simulink model "ADCSSimulator"  (R2024a)
settings: Solver=ode4  StartTime=0.0  StopTime=600  FixedStep=0.01  MaxStep=0.1  RelTol=1e-3  AbsTol=1e-3
values from neighbouring files (symbols this model uses):
  ActuatorAllocationMatrix = ActuatorPhysicalMatrix' * inv(ActuatorPhysicalMatrix * ActuatorPhysicalMatrix')    [set_Init.m]
  ActuatorPhysicalMatrix = [1, 0, 0, 0 ... (first row only)    [set_Init.m]
  albedo_irradiance = 300    [set_Init.m]
  b = 0    [set_Init.m]
  Cd = 2.2    [set_Init.m]
  h_bias = [0; 0; 0]    [set_Init.m]
  J = 4.0e-3 / 628    (= 6.36942675159e-06)    [set_Init.m]
  k_Bdot = ((4 * pi * 0.5236 * 0.0055) / (5677.2 * (4.5e-5)^2))    (= 3147.8423197)    [set_Init.m]
  K_E = K_T    (= 0.0022)    [set_Init.m]
  K_T = 0.0022    [set_Init.m]
  P0 = blkdiag(P0_att, P0_bias)    [set_Init.m]
  P0_att = eye(3) * initial_variance_rad2    [set_Init.m]
  PowerVoltageBus_01 = 3.3    [set_Init.m]
  PowerVoltageBus_02 = 3.3    [set_Init.m]
  PowerVoltageBus_03 = 3.3    [set_Init.m]
  PowerVoltageBus_04 = 3.3    [set_Init.m]
  PowerVoltageBus_05 = 3.3    [set_Init.m]
  PowerVoltageBus_06 = 3.3    [set_Init.m]
  PowerVoltageBus_07 = 3.3    [set_Init.m]
  PowerVoltageBus_08 = 3.3    [set_Init.m]
  PowerVoltageBus_09 = 3.3    [set_Init.m]
  PowerVoltageBus_10 = 3.3    [set_Init.m]
  PowerVoltageBus_11 = 3.3    [set_Init.m]
  PowerVoltageBus_12 = 0.0    (= 0)    [set_Init.m]
  PowerVoltageBus_13 = 0.0    (= 0)    [set_Init.m]
  PowerVoltageBus_14 = 0.0    (= 0)    [set_Init.m]
  PowerVoltageBus_15 = 0.0    (= 0)    [set_Init.m]
  R = 2.0    (= 2)    [set_Init.m]
  ressidual_m = [3e-4; -2e-4; 1e-4]    [set_Init.m]
  solar_irradiance = 1361    [set_Init.m]
  surface_areas = [A_xy, A_yz, A_xz, A_xy, A_yz, A_xz]    [set_Init.m]
  surface_normals_body = [eye(3) -eye(3)]    [set_Init.m]
  surface_positions_body = [       hx,   0,   0 ... (first row only)    [set_Init.m]
  surface_reflectivities = [0.9 0.8 0.9 0.9 0.9 0.9]    [set_Init.m]
  Switch_01 = 1    [set_Init.m]
  Switch_02 = 1    [set_Init.m]
  Switch_03 = 1    [set_Init.m]
  Switch_04 = 1    [set_Init.m]
  Switch_05 = 1    [set_Init.m]
  Switch_06 = 1    [set_Init.m]
  Switch_07 = 1    [set_Init.m]
  Switch_08 = 1    [set_Init.m]
  Switch_09 = 1    [set_Init.m]
  Switch_10 = 1    [set_Init.m]
  Switch_11 = 1    [set_Init.m]
  Switch_12 = 0    [set_Init.m]
  Switch_13 = 0    [set_Init.m]
  Switch_14 = 0    [set_Init.m]
  Switch_15 = 0    [set_Init.m]
  visSampleTime = 0.1    [set_Init.m]
undefined symbols (not defined in the file or in its folder): attitude, Controller, epoch, IAU, juliandate, Kd, km, Kp, m, rad, s, satellite, SGP4_parameters, simulator, UKF_parameters, WMM2020
libraries: sharedtransform x27, aerolibutil x22, aerolibconvert2 x18, simulink_extras x16, matrix_library x6, aerolibtransform2 x4, vrlib x2, aerolibgravity2 x2, aerolibobsolete x1, aerolibattitudesys x1, simulink x1
(part 3 of 8)

== system ADCSSimulator/ADCS/ADCS Hardware/Actuators/Tri-axial Magnetorquer Model (MTQs) ==
  Magnetic Field [Body] (T) : Inport
  MTQ CMD (A.m^2) : Inport  Port=2  PortDimensions=[3,1]
  Bus Voltage : Inport  Port=3
  Abs : Abs  SaturateOnIntegerOverflow=off
  Abs1 : Abs  SaturateOnIntegerOverflow=off
  Bus Creator : BusCreator  Inputs=3
  Bus Selector : BusSelector  OutputSignals=Power Bus: MTQ_X (signal 9),Power Bus: MTQ_Y (signal 10),Power Bus: MTQ_Z (signal 11)
  Constant : Constant  Value=[1;1;1]
  Constant1 : Constant  Value=[1;1;1]
  Cross Product : vrlib/Utilities/Cross Product
  Demux : Demux  Outputs=3
  Gain : Gain  Gain=0.5
  Gain1 : Gain  Gain=-1
  Gain2 : Gain  Gain=0.5
  Magnetorquers Bus Creator : BusCreator  Inputs=3
  Mux : Mux  Inputs=3
  Nominal Dipole : Constant  Value=satellite.MTQ.DPMoment
  Power Consumption Calculator : Subsystem
  Power Consumption Calculator1 : Subsystem
  Power Consumption Calculator2 : Subsystem
  Product : Product  Inputs=3
  Product1 : Product  Inputs=*/
  Product2 : Product
  Product3 : Product
  Sign{,1..3} (4 alike) : Signum
  Sum : Sum  Inputs=|+-
  Sum1 : Sum  Inputs=|++
  Sum2 : Sum  Inputs=|++
  Sum3 : Sum  Inputs=|++
  maximum allowable magnetic dipole moment : Constant  Value=satellite.MTQ.DPMoment
  Acutators: MTQs : Outport
  wires:
  Product3/1 -> Abs/1, Product2/1, Sign1/1, Product1/1  "m_mod"
  Product2/1 -> Sum3/1
  Product1/1 -> Abs1/1
  Gain/1 -> Product/2  "1: |m_mod| > m_max"
  Abs1/1 -> Demux/1
  Product/1 -> Sum3/2
  Sum1/1 -> Gain/1  "2: |m_mod| > m_max"
  Nominal Dipole/1 -> Sum/2, Product/3  "m_max"
  Sign/1 -> Sum1/1  "1: |m_mod| > m_max"
  Bus Creator/1 -> Magnetorquers Bus Creator/3  "MTQs Power Status"
  Magnetic Field [Body] (T)/1 -> Cross Product/2
  Gain2/1 -> Product2/2  "1: m_max > |m_mod|"
  Sum3/1 -> Magnetorquers Bus Creator/1, Cross Product/1  "Dipoles (Am^2)"
  maximum allowable magnetic dipole moment/1 -> Product1/2
  Sum2/1 -> Gain2/1  "2: m_max > |m_mod|"
  Sign2/1 -> Sum2/1  "1: m_max > |m_mod|"
  Constant1/1 -> Sum2/2
  Sum/1 -> Gain1/1, Sign/1
  MTQ CMD (A.m^2)/1 -> Product3/1
  Magnetorquers Bus Creator/1 -> Acutators: MTQs/1  "Actuators"
  Constant/1 -> Sum1/2
  Cross Product/1 -> Magnetorquers Bus Creator/2  "MTQs Torque [Body] (Nm)"
  Sign1/1 -> Product/1
  Gain1/1 -> Sign2/1  "m_max - |m_mod|"
  Abs/1 -> Sum/1  "|m_mod|"
  Power Consumption Calculator2/1(Power Consumption) -> Bus Creator/1  "Power Consumption [Magnetorquer X]"
  Power Consumption Calculator/1(Power Consumption) -> Bus Creator/3  "Power Consumption [Magnetorquer Z]"
  Power Consumption Calculator1/1(Power Consumption) -> Bus Creator/2  "Power Consumption [Magnetorquer Y]"
  Sign3/1 -> Product3/2  "MTQ Switches"
  [InputVoltage] -> Sign3/1
  Demux/1 -> [DipoleRatioX]  "|m/m_max| (X)"
  Demux/2 -> [DipoleRatioY]  "|m/m_max| (Y)"
  Demux/3 -> [DipoleRatioZ]  "|m/m_max| (Z)"
  [DipoleRatioX] -> Power Consumption Calculator2/2(|m/m_max|)
  [DipoleRatioY] -> Power Consumption Calculator1/2(|m/m_max|)
  [DipoleRatioZ] -> Power Consumption Calculator/2(|m/m_max|)
  Bus Voltage/1 -> Bus Selector/1
  Mux/1 -> [InputVoltage]
  Bus Selector/1 -> Mux/1, Power Consumption Calculator2/1(Bus Voltage (V))  "<Power Bus: MTQ_X (signal 9)>"
  Bus Selector/2 -> Mux/2, Power Consumption Calculator1/1(Bus Voltage (V))  "<Power Bus: MTQ_Y (signal 10)>"
  Bus Selector/3 -> Mux/3, Power Consumption Calculator/1(Bus Voltage (V))  "<Power Bus: MTQ_Z (signal 11)>"

== system ADCSSimulator/ADCS/ADCS Hardware/Sensors/Analog Magnetometer Model ==
  note: sensivity is used for analog magnetometer
  Magnetic Field [Body] (T) : Inport
  Temperature (˚C) : Inport  Port=2
  Input Voltage (V) : Inport  Port=3
  Measurement Model DCM : Inport  Port=4
  Constant1 : Constant  Value=[1e-4, 1e-4,1e-4]
  Gain3 : Gain  Gain=10^-9
  Init Data Wrapper : Subsystem
  MATLAB Function : MATLAB Function  Commented=on  TreatAsAtomicUnit=on
  Matrix Multiply : Product  Multiplication=Matrix(*)
  Noise : RandomNumber  Variance=satellite.MM.NoiseVariance  SampleTime=1/satellite.MM.Frequency
  Nominal Temperature (˚C) : Constant  Value=20
  Offset (nT) : Constant  Value=satellite.MM.ZeroFieldBias*satellite.MM.Sensitivity
  Power Consumption Calculator : Subsystem
  Product : Product  Inputs=3
  Product1 : Product
  Product2 : Product
  Product4 : Product
  Quantization : Quantizer  QuantizationInterval=satellite.MM.QuantizationInterval
  Saturation : Saturate  UpperLimit=satellite.MM.Range(2)  LowerLimit=satellite.MM.Range(1)
  Scale Factor Drift : Constant  Value=satellite.MM.ScaleFactorDrift*1e-6
  Scale error : Constant  Value=satellite.MM.Accuracy*1e-2
  Sensivity : Gain  Gain=satellite.MM.Sensitivity
  Sign : Signum
  Sum : Sum  Inputs=+++++
  Sum1 : Sum  Inputs=++|
  Sum2 : Sum  Inputs=|+-
  Sum3 : Sum  Inputs=++|
  T to nT : Gain  Gain=10^9
  Unit Delay4 : UnitDelay  SampleTime=-1  HasFrameUpgradeWarning=on
  Zero Field Bias (nT) : Constant  Value=satellite.MM.ZeroFieldBias
  Zero Field Drift : Constant  Value=satellite.MM.ZeroFieldDrift
  Zero-Order Hold : ZeroOrderHold  SampleTime=1/satellite.MM.Frequency
  Measured Magnetic Field [Body] (T) : Outport  PortDimensions=[3,1]
  Power Consumption : Outport  Port=2
  wires:
  Zero Field Bias (nT)/1 -> Sum3/1
  T to nT/1 -> Sum3/2
  Quantization/1 -> Init Data Wrapper/1(Real Data)
  Init Data Wrapper/1(Wrapped Data) -> Measured Magnetic Field [Body] (T)/1
  Constant1/1 -> Init Data Wrapper/2(Initial Value)
  [InputVoltage] -> Sign/1
  Power Consumption Calculator/1(MM Power Consumption) -> Power Consumption/1  "Magnetometer Power Consumption"
  Matrix Multiply/1 -> T to nT/1
  Unit Delay4/1 -> Product4/2
  Gain3/1 -> Product4/1
  Magnetic Field [Body] (T)/1 -> Matrix Multiply/2
  Sensivity/1 -> Sum1/2
  Sum1/1 -> Saturation/1
  Sum3/1 -> Sum/2, Product/1, Product1/2  "Magnetic Field [Sensor] (nT)"
  Noise/1 -> Sum/5
  Scale Factor Drift/1 -> Product/2
  Product4/1 -> Quantization/1  "Magnetic Field [Sensor] (T)"
  Zero Field Drift/1 -> Product2/2
  Sum/1 -> Sensivity/1
  Input Voltage (V)/1 -> Power Consumption Calculator/1(Bus Voltage (V)), [InputVoltage]
  Sign/1 -> Unit Delay4/1  "Sensor Switch"
  Product1/1 -> Sum/1
  Product/1 -> Sum/3
  Temperature (˚C)/1 -> Sum2/1
  Measurement Model DCM/1 -> Matrix Multiply/1
  Offset (nT)/1 -> Sum1/1
  Nominal Temperature (˚C)/1 -> Sum2/2
  Zero-Order Hold/1 -> Gain3/1
  Product2/1 -> Sum/4
  Saturation/1 -> Zero-Order Hold/1
  Sum2/1 -> Product2/1, Product/3
  Scale error/1 -> Product1/1

== system ADCSSimulator/ADCS/ADCS Hardware/Sensors/Digital Magnetometer Model ==
  Magnetic Field [Body] (T) : Inport
  Temperature (˚C) : Inport  Port=2
  Input Voltage (V) : Inport  Port=3
  Measurement Model DCM : Inport  Port=4
  Constant1 : Constant  Value=[1e-4, 1e-4,1e-4]
  Gain3 : Gain  Gain=10^-9
  Init Data Wrapper : Subsystem
  Matrix Multiply : Product  Multiplication=Matrix(*)
  Noise : RandomNumber  Variance=satellite.MM.NoiseVariance  SampleTime=1/satellite.MM.Frequency
  Nominal Temperature (˚C) : Constant  Value=20
  Onboard Disturbance Bias (nT) : Constant  Value=satellite.MM.OnboardDistBias
  Power Consumption Calculator : Subsystem
  Product : Product  Inputs=3
  Product1 : Product
  Product2 : Product
  Product4 : Product
  Quantization : Quantizer  QuantizationInterval=satellite.MM.QuantizationInterval
  Saturation : Saturate  UpperLimit=satellite.MM.Range(2)  LowerLimit=satellite.MM.Range(1)
  Scale Factor Drift : Constant  Value=satellite.MM.ScaleFactorDrift*1e-6
  Scale error : Constant  Value=satellite.MM.Accuracy*1e-2
  Sign : Signum
  Sum : Sum  Inputs=+++++++
  Sum2 : Sum  Inputs=|+-
  T to nT : Gain  Gain=10^9
  Unit Delay4 : UnitDelay  SampleTime=-1  HasFrameUpgradeWarning=on
  Zero Field Bias (nT) : Constant  Value=satellite.MM.ZeroFieldBias
  Zero Field Drift : Constant  Value=satellite.MM.ZeroFieldDrift
  Zero-Order Hold : ZeroOrderHold  SampleTime=1/satellite.MM.Frequency
  Measured Magnetic Field [Body] (T) : Outport  PortDimensions=[3,1]
  Power Consumption : Outport  Port=2
  wires:
  Scale error/1 -> Product1/1
  Sum2/1 -> Product2/1, Product/3
  Product2/1 -> Sum/4
  Nominal Temperature (˚C)/1 -> Sum2/2
  Measurement Model DCM/1 -> Matrix Multiply/1
  Temperature (˚C)/1 -> Sum2/1
  Product/1 -> Sum/3
  Product1/1 -> Sum/1
  Sign/1 -> Unit Delay4/1  "Sensor Switch"
  Input Voltage (V)/1 -> [InputVoltage], Power Consumption Calculator/1(Bus Voltage (V))
  Zero Field Drift/1 -> Product2/2
  Product4/1 -> Init Data Wrapper/1(Real Data)  "Magnetic Field [Sensor] (T)"
  Scale Factor Drift/1 -> Product/2
  Noise/1 -> Sum/7
  T to nT/1 -> Product/1, Sum/2, Product1/2  "Magnetic Field [Sensor] (nT)"
  Sum/1 -> Saturation/1
  Magnetic Field [Body] (T)/1 -> Matrix Multiply/2
  Gain3/1 -> Product4/1
  Unit Delay4/1 -> Product4/2
  Matrix Multiply/1 -> T to nT/1
  Power Consumption Calculator/1(MM Power Consumption) -> Power Consumption/1  "Magnetometer Power Consumption"
  [InputVoltage] -> Sign/1
  Constant1/1 -> Init Data Wrapper/2(Initial Value)
  Init Data Wrapper/1(Wrapped Data) -> Measured Magnetic Field [Body] (T)/1
  Quantization/1 -> Zero-Order Hold/1
  Zero Field Bias (nT)/1 -> Sum/5
  Onboard Disturbance Bias (nT)/1 -> Sum/6
  Saturation/1 -> Quantization/1
  Zero-Order Hold/1 -> Gain3/1

== system ADCSSimulator/ADCS/ADCS Hardware/Sensors/GNSS Receiver Model ==
  Calendar : Inport
  ICRF to ITRF TM : Inport  Port=2
  Satellite Ephemeris : Inport  Port=3
  " Input Voltage (V)" : Inport  Port=4
  Bus Selector1 : BusSelector  OutputSignals=Julian Date (day)
  Bus Selector7 : BusSelector  OutputSignals=Satellite Position [ICRF](m),Satellite Velocity [ICRF](m/s)
  Constant : Constant  Value=satellite.GPS.Position.Bias
  Constant1 : Constant  Value=satellite.GPS.Velocity.Bias
  Gauss-Markov : Subsystem
  Gauss-Markov1 : Subsystem
  Gauss-Markov2 : Subsystem
  Gauss-Markov3 : Subsystem
  Gauss-Markov4 : Subsystem
  Gauss-Markov5 : Subsystem
  ICRF to ITRF TM1 : InportShadow  Port=2
  Matrix Multiply : Product  Multiplication=Matrix(*)
  Matrix Multiply1 : Product  Multiplication=Matrix(*)
  Measured Eph. Bus Creator : BusCreator  Inputs=3
  Mux3 : Mux  Inputs=3
  Mux4 : Mux  Inputs=3
  Power Consumption Calculator : Subsystem
  Product1 : Product
  Product2 : Product
  Product8 : Product
  Quantizer : Quantizer  QuantizationInterval=satellite.GPS.Position.QuantizationInterval
  Quantizer1 : Quantizer  QuantizationInterval=satellite.GPS.Velocity.QuantizationInterval
  Sign : Signum
  Sum2 : Sum  Inputs=+++
  Sum8 : Sum  Inputs=+++
  Unit Delay1 : UnitDelay  SampleTime=-1  HasFrameUpgradeWarning=on
  Zero-Order Hold2 : ZeroOrderHold  SampleTime=1/satellite.GPS.Frequency
  Zero-Order Hold3 : ZeroOrderHold  SampleTime=1/satellite.GPS.Frequency
  Zero-Order Hold4 : ZeroOrderHold  SampleTime=1/satellite.GPS.Frequency
  Measured Satellite Ephemeris : Outport
  Power Consumption : Outport  Port=2
  wires:
  Product1/1 -> Measured Eph. Bus Creator/1  "Julian Date (day)"
  Gauss-Markov1/1(Correlated Noise Out) -> Mux4/2
  Sum8/1 -> Zero-Order Hold4/1  "Measured Velocity [ITRF] (m/s)"
  Sign/1 -> Unit Delay1/1  "Sensor Switch"
  Zero-Order Hold3/1 -> Quantizer/1
  Product8/1 -> Measured Eph. Bus Creator/3  "Measured Velocity [ITRF] (m/s)"
  Measured Eph. Bus Creator/1 -> Measured Satellite Ephemeris/1  "Measured Ephemeris"
  Zero-Order Hold2/1 -> Product1/1
  Unit Delay1/1 -> Product8/2, Product2/2, Product1/2
  Product2/1 -> Measured Eph. Bus Creator/2  "Measured Position [ITRF] (m)"
  Power Consumption Calculator/1(GPS Power Consumption) -> Power Consumption/1  "GPS Power Consumption"
  Gauss-Markov5/1(Correlated Noise Out) -> Mux3/1
  Bus Selector7/1 -> Matrix Multiply/2  "<Satellite Position [ICRF](m)>"
  Zero-Order Hold4/1 -> Quantizer1/1
  Bus Selector7/2 -> Matrix Multiply1/2  "<Satellite Velocity [ICRF](m/s)>"
  " Input Voltage (V)"/1 -> [InputVoltage], Power Consumption Calculator/1(Bus Voltage (V))
  Sum2/1 -> Zero-Order Hold3/1  "Measured Position [ITRF] (m)"
  Mux3/1 -> Sum2/3
  Gauss-Markov4/1(Correlated Noise Out) -> Mux3/2
  Mux4/1 -> Sum8/3
  Gauss-Markov3/1(Correlated Noise Out) -> Mux3/3
  Gauss-Markov2/1(Correlated Noise Out) -> Mux4/3
  Bus Selector1/1 -> Zero-Order Hold2/1  "<Julian Date (day)>"
  Satellite Ephemeris/1 -> Bus Selector7/1
  Calendar/1 -> Bus Selector1/1
  Gauss-Markov/1(Correlated Noise Out) -> Mux4/1
  [InputVoltage] -> Sign/1
  Constant/1 -> Sum2/1
  Constant1/1 -> Sum8/1
  Quantizer/1 -> Product2/1
  Quantizer1/1 -> Product8/1
  ICRF to ITRF TM/1 -> Matrix Multiply/1
  Matrix Multiply/1 -> Sum2/2  "Satellite Position [ITRF] (m)"
  Matrix Multiply1/1 -> Sum8/2  "Satellite Velocity [ITRF] (m/s)"
  ICRF to ITRF TM1/1 -> Matrix Multiply1/1

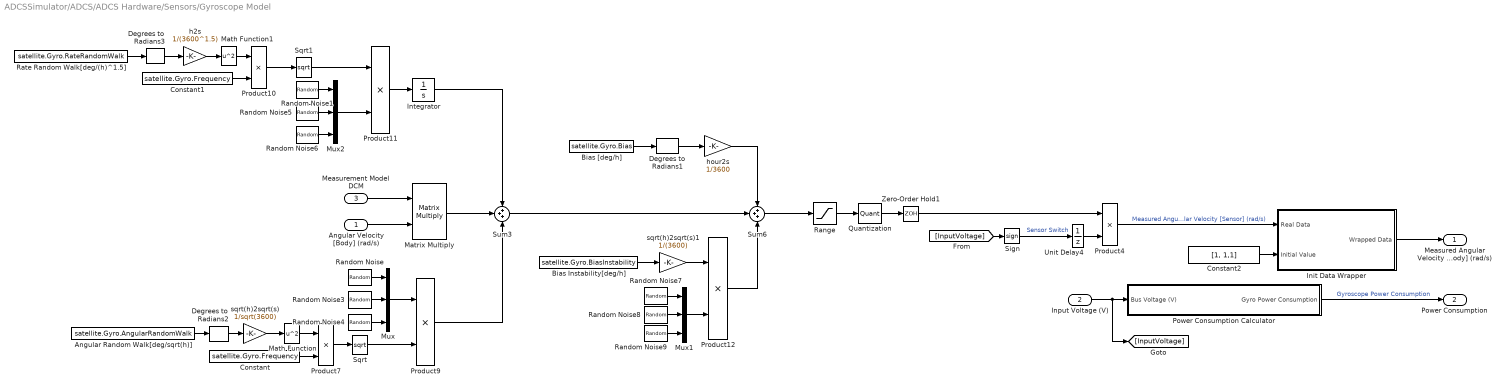
== system ADCSSimulator/ADCS/ADCS Hardware/Sensors/Gyroscope Model ==
  Angular Velocity [Body] (rad/s) : Inport
  Input Voltage (V) : Inport  Port=2
  Measurement Model DCM : Inport  Port=3
  Angular Random Walk[deg/sqrt(h)] : Constant  Value=satellite.Gyro.AngularRandomWalk
  Bias Instability[deg/h] : Constant  Value=satellite.Gyro.BiasInstability
  Bias [deg/h] : Constant  Value=satellite.Gyro.Bias
  Constant : Constant  Value=satellite.Gyro.Frequency
  Constant1 : Constant  Value=satellite.Gyro.Frequency
  Constant2 : Constant  Value=[1, 1,1]
  Degrees to Radians1 : simulink_extras/Transformations/Degrees to Radians
  Degrees to Radians2 : simulink_extras/Transformations/Degrees to Radians
  Degrees to Radians3 : simulink_extras/Transformations/Degrees to Radians
  Init Data Wrapper : Subsystem
  Integrator : Integrator  InitialCondition=[0;0;0]
  Math Function : Math  Operator=square  SignedPower=on
  Math Function1 : Math  Operator=square  SignedPower=on
  Matrix Multiply : Product  Multiplication=Matrix(*)
  Mux : Mux  Inputs=3
  Mux1 : Mux  Inputs=3
  Mux2 : Mux  Inputs=3
  Power Consumption Calculator : Subsystem
  Product{4,7,9..12} (6 alike) : Product
  Quantization : Quantizer  QuantizationInterval=satellite.Gyro.QuantizationInterval
  Random Noise{,1,3..9} (9 alike) : RandomNumber  SampleTime=1/satellite.Gyro.Frequency
  Range : Saturate  UpperLimit=satellite.Gyro.Range(2)  LowerLimit=satellite.Gyro.Range(1)
  Rate Random Walk[deg/(h)^1.5] : Constant  Value=satellite.Gyro.RateRandomWalk
  Sign : Signum
  Sqrt : Sqrt
  Sqrt1 : Sqrt
  Sum3 : Sum  Inputs=+++
  Sum6 : Sum  Inputs=+++
  Unit Delay4 : UnitDelay  SampleTime=-1  HasFrameUpgradeWarning=on
  Zero-Order Hold1 : ZeroOrderHold  SampleTime=1/satellite.Gyro.Frequency
  h2s : Gain  Gain=1/(3600^1.5)
  hour2s : Gain  Gain=1/3600
  sqrt(h)2sqrt(s) : Gain  Gain=1/sqrt(3600)
  sqrt(h)2sqrt(s)1 : Gain  Gain=1/(3600)
  Measured Angular Velocity [Body] (rad/s) : Outport  PortDimensions=[3,1]
  Power Consumption : Outport  Port=2
  wires:
  Sqrt/1 -> Product9/2
  Matrix Multiply/1 -> Sum3/2
  hour2s/1 -> Sum6/1
  Range/1 -> Quantization/1
  Random Noise3/1 -> Mux/2
  Mux/1 -> Product9/1
  Degrees to Radians3/1 -> h2s/1
  Product12/1 -> Sum6/3
  Product9/1 -> Sum3/3
  Product10/1 -> Sqrt1/1
  Random Noise5/1 -> Mux2/2
  Sum3/1 -> Sum6/2
  Integrator/1 -> Sum3/1
  Random Noise6/1 -> Mux2/3
  Math Function/1 -> Product7/1
  sqrt(h)2sqrt(s)/1 -> Math Function/1
  Mux2/1 -> Product11/2
  Sum6/1 -> Range/1
  Angular Velocity [Body] (rad/s)/1 -> Matrix Multiply/2
  Constant/1 -> Product7/2
  Bias Instability[deg/h]/1 -> sqrt(h)2sqrt(s)1/1
  Random Noise4/1 -> Mux/3
  Angular Random Walk[deg/sqrt(h)]/1 -> Degrees to Radians2/1
  Random Noise/1 -> Mux/1
  Rate Random Walk[deg/(h)^1.5]/1 -> Degrees to Radians3/1
  Measurement Model DCM/1 -> Matrix Multiply/1
  Math Function1/1 -> Product10/1
  h2s/1 -> Math Function1/1
  Constant1/1 -> Product10/2
  Product7/1 -> Sqrt/1
  Zero-Order Hold1/1 -> Product4/1
  Sqrt1/1 -> Product11/1
  Product11/1 -> Integrator/1
  [InputVoltage] -> Sign/1
  sqrt(h)2sqrt(s)1/1 -> Product12/1
  Bias [deg/h]/1 -> Degrees to Radians1/1
  Degrees to Radians2/1 -> sqrt(h)2sqrt(s)/1
  Product4/1 -> Init Data Wrapper/1(Real Data)  "Measured Angular Velocity [Sensor] (rad/s)"
  Degrees to Radians1/1 -> hour2s/1
  Random Noise1/1 -> Mux2/1
  Input Voltage (V)/1 -> [InputVoltage], Power Consumption Calculator/1(Bus Voltage (V))
  Unit Delay4/1 -> Product4/2
  Power Consumption Calculator/1(Gyro Power Consumption) -> Power Consumption/1  "Gyroscope Power Consumption"
  Sign/1 -> Unit Delay4/1  "Sensor Switch"
  Constant2/1 -> Init Data Wrapper/2(Initial Value)
  Init Data Wrapper/1(Wrapped Data) -> Measured Angular Velocity [Body] (rad/s)/1
  Quantization/1 -> Zero-Order Hold1/1
  Random Noise8/1 -> Mux1/2
  Mux1/1 -> Product12/2
  Random Noise7/1 -> Mux1/1
  Random Noise9/1 -> Mux1/3

== system ADCSSimulator/ADCS/ADCS Hardware/Sensors/Sun Sensor Model ==
  Eclipse : Inport
  q [ICRF to Body] : Inport  Port=2
  Sun Position [ICRF] (m) : Inport  Port=3
  Input Voltage (V) : Inport  Port=4
  Bias: Misalagnment Matrix in Body Frame : Constant  Value=satellite.SS.MisalagnmentMatrix
  Cartesian to Spherical : simulink_extras/Transformations/Cartesian to Spherical
  Constant1 : Constant  Value=[1,1,1]
  Demux4 : Demux  Outputs=3
  Eclipse=1 (Sun vector is not available) : Constant  Value=0
  Init Data Wrapper : Subsystem
  Matrix Multiply : Product  Multiplication=Matrix(*)
  Mux2 : Mux  Inputs=3
  Normalizer8 : Subsystem
  Output NaN in Eclipse : MATLAB Function  TreatAsAtomicUnit=on
  Power Consumption Calculator : Subsystem
  Product : Product
  Quantization : Quantizer  QuantizationInterval=satellite.SS.QuantizationInterval
  Quaternion Rotation : aerolibutil/Quaternion Rotation
  Random Noise (Phi) : RandomNumber  Variance=(satellite.SS.AngularNoise_RMS * pi/180)^2  SampleTime=1/satellite.SS.Frequency
  Random Noise (Theta) : RandomNumber  Variance=(satellite.SS.AngularNoise_RMS * pi/180)^2  SampleTime=1/satellite.SS.Frequency
  Sign : Signum
  Spherical to Cartesian : simulink_extras/Transformations/Spherical to Cartesian
  Sum10 : Sum  Inputs=|++
  Sum11 : Sum  Inputs=|++
  Switch : Switch  Criteria=u2 > Threshold  SaturateOnIntegerOverflow=off  InputSameDT=off
  Unit Delay : UnitDelay  SampleTime=-1  HasFrameUpgradeWarning=on
  Zero-Order Hold2 : ZeroOrderHold  SampleTime=1/satellite.SS.Frequency
  Measured Sun Vector [Body] (m) : Outport
  Power Consumption : Outport  Port=2
  wires:
  Zero-Order Hold2/1 -> Product/1  "Staircase Sun Vector Signal"
  Random Noise (Theta)/1 -> Sum10/2
  Spherical to Cartesian/3 -> Mux2/3
  Demux4/1 -> Cartesian to Spherical/1
  Spherical to Cartesian/2 -> Mux2/2
  Cartesian to Spherical/1 -> Spherical to Cartesian/1
  Demux4/2 -> Cartesian to Spherical/2
  Eclipse=1 (Sun vector is not available)/1 -> Switch/1
  Spherical to Cartesian/1 -> Mux2/1
  Mux2/1 -> Switch/3
  Sum10/1 -> Spherical to Cartesian/2
  Sum11/1 -> Spherical to Cartesian/3
  Cartesian to Spherical/2 -> Sum10/1
  Random Noise (Phi)/1 -> Sum11/2
  Demux4/3 -> Cartesian to Spherical/3
  Sun Position [ICRF] (m)/1 -> Quaternion Rotation/2
  Switch/1 -> Quantization/1
  Cartesian to Spherical/3 -> Sum11/1
  Quaternion Rotation/1 -> Normalizer8/1(A)  "True Sun Position [Body] (m)"
  q [ICRF to Body]/1 -> Quaternion Rotation/1
  Power Consumption Calculator/1(SS Power Consumption) -> Power Consumption/1
  Product/1 -> Init Data Wrapper/1(Real Data)
  Input Voltage (V)/1 -> [InputVoltage], Power Consumption Calculator/1(Bus Voltage (V))
  Sign/1 -> Unit Delay/1  "Sensor Switch"
  Unit Delay/1 -> Product/2
  [InputVoltage] -> Sign/1
  Eclipse/1 -> Switch/2
  Constant1/1 -> Init Data Wrapper/2(Initial Value)
  Init Data Wrapper/1(Wrapped Data) -> Output NaN in Eclipse/1(u)
  Quantization/1 -> Zero-Order Hold2/1
  Matrix Multiply/1 -> Demux4/1  "Biased Sun Vector [Body] (m)"
  Bias: Misalagnment Matrix in Body Frame/1 -> Matrix Multiply/1
  Output NaN in Eclipse/1(y) -> Measured Sun Vector [Body] (m)/1  "V_2"
  Normalizer8/1(Normalized(A)) -> Matrix Multiply/2  "True Sun Vector [Body] (m)"

== system ADCSSimulator/ADCS/ADCS Software/Attitude Control/Chart/Detumbling ==
  MeasuredAngularVelocity_Body : Inport
  MeasuredMagneticField_Body : Inport  Port=2
  Action Port : ActionPort
      settings: CopyFcn=Stateflow.SLINSF.SimulinkMan.removeBlockPreDeleteFcn  PreDeleteFcn=Stateflow.SLINSF.SimulinkMan.unsafePredeleteFcn
  Constant : Constant  Value=[0; 0; 0]
  Cross Product : matrix_library/Cross Product
  Detumbling Algorithm : Subsystem  TreatAsAtomicUnit=on
  Manual Switch : ManualSwitch
  Manual Switch1 : ManualSwitch
  TorqueCommand : Outport
  DipoleCommand : Outport  Port=2
  wires:
  Manual Switch1/1 -> DipoleCommand/1  "Detumbling Command"
  Manual Switch/1 -> TorqueCommand/1
  MeasuredMagneticField_Body/1 -> [B_Body], Detumbling Algorithm/1(Measured Magnetic Field [Body](T))
  MeasuredAngularVelocity_Body/1 -> Detumbling Algorithm/2(Measured Angular Velocity [Body](rad/s))
  Detumbling Algorithm/1(Detumbling: Magnetic Dipole Command) -> Manual Switch1/1, Cross Product/1
  Constant/1 -> Manual Switch1/2, Manual Switch/1
  Cross Product/1 -> Manual Switch/2
  [B_Body] -> Cross Product/2

== system ADCSSimulator/ADCS/ADCS Software/Attitude Control/Chart/Nadir_Pointing ==
  MeasuredMagneticField_Body : Inport
  qDesired_NadirPointing : Inport  Port=2
  MeasuredAngularVelocity_Body : Inport  Port=3
  ICRF2BodyQuaternions : Inport  Port=4
  Wheel_Momentum_Vector : Inport  Port=5
  Action Port : ActionPort
      settings: CopyFcn=Stateflow.SLINSF.SimulinkMan.removeBlockPreDeleteFcn  PreDeleteFcn=Stateflow.SLINSF.SimulinkMan.unsafePredeleteFcn
  Actuator Allocation & Feed-Forward : Subsystem
  MeasuredMagneticField_Body1 : InportShadow
  MeasuredMagneticField_Body2 : InportShadow
  Momentum Management : Subsystem
  Quaternion Inverse : aerolibutil/Quaternion Inverse
  Terminator : Terminator
  َAttitude Controller (LQR Controller) : Subsystem
  DipoleCommand : Outport
  TorqueCommand : Outport  Port=2
  ErrorQuaternion : Outport  Port=3
  wires:
  qDesired_NadirPointing/1 -> َAttitude Controller (LQR Controller)/3(Desired Quaternion)
  MeasuredMagneticField_Body/1 -> َAttitude Controller (LQR Controller)/4(MagneticField [Body])
  َAttitude Controller (LQR Controller)/2(Nadir Pointing: Torque Command) -> [tau_req]  "Nadir Pointing: Torque Command"
  َAttitude Controller (LQR Controller)/1(Nadir Pointing: Magnetic Dipole Command) -> Terminator/1  "Nadir Pointing: Magnetic Dipole Command from Torque"
  MeasuredAngularVelocity_Body/1 -> َAttitude Controller (LQR Controller)/1(AngularVelocity [Body])
  ICRF2BodyQuaternions/1 -> Quaternion Inverse/1
  Quaternion Inverse/1 -> َAttitude Controller (LQR Controller)/2(Body to ICRF Quaternion)
  MeasuredMagneticField_Body1/1 -> Momentum Management/2(B_meas_Body_T)
  َAttitude Controller (LQR Controller)/3(Error Quaternion) -> ErrorQuaternion/1
  Wheel_Momentum_Vector/1 -> Momentum Management/1(h_rw_Nms)
  Momentum Management/1(m_cmd_raw_Am2) -> [m_cmd_raw]
  Actuator Allocation & Feed-Forward/1(m_cmd_final) -> DipoleCommand/1
  Actuator Allocation & Feed-Forward/2(tau_rw_cmd) -> TorqueCommand/1
  [tau_req] -> Actuator Allocation & Feed-Forward/2(tau_req_Nm)
  [m_cmd_raw] -> Actuator Allocation & Feed-Forward/1(m_cmd_raw_Am2)
  MeasuredMagneticField_Body2/1 -> Actuator Allocation & Feed-Forward/3(B_meas_Body_T)

== system ADCSSimulator/ADCS/ADCS Software/Attitude Control/Chart/Off ==
  Action Port : ActionPort
      settings: CopyFcn=Stateflow.SLINSF.SimulinkMan.removeBlockPreDeleteFcn  PreDeleteFcn=Stateflow.SLINSF.SimulinkMan.unsafePredeleteFcn
  Constant : Constant  Value=[0; 0; 0]
  Constant1 : Constant  Value=[0; 0; 0]
  TorqueCommand : Outport
  DipoleCommand : Outport  Port=2
  wires:
  Constant1/1 -> DipoleCommand/1
  Constant/1 -> TorqueCommand/1

== system ADCSSimulator/ADCS/ADCS Software/Attitude Control/Chart/Sun_Pointing ==
  MeasuredAngularVelocity_Body : Inport
  MeasuredMagneticField_Body : Inport  Port=2
  ICRF2BodyQuaternions : Inport  Port=3
  qDesired_SunPointing : Inport  Port=4
  Wheel_Momentum_Vector : Inport  Port=5
  Action Port : ActionPort
      settings: CopyFcn=Stateflow.SLINSF.SimulinkMan.removeBlockPreDeleteFcn  PreDeleteFcn=Stateflow.SLINSF.SimulinkMan.unsafePredeleteFcn
  Sun Pointing Algorithm (LQR) : Subsystem
  Sun Pointing Algorithm (PD) : Subsystem  Commented=on
  TorqueCommand : Outport
  DipoleCommand : Outport  Port=2
  ErrorQuaternion : Outport  Port=3
  wires:
  ICRF2BodyQuaternions/1 -> Sun Pointing Algorithm (LQR)/3(ICRF to Body Quaternions)
  Sun Pointing Algorithm (LQR)/1(Sun Pointing: Magnetic Dipole Command) -> DipoleCommand/1  "Sun Pointing: Magnetic Dipole Command"
  Sun Pointing Algorithm (LQR)/2(Sun Pointing: Torque Command) -> TorqueCommand/1  "Sun Pointing: Torque Command"
  MeasuredAngularVelocity_Body/1 -> Sun Pointing Algorithm (LQR)/1(Angular Velocity [Body] (T))
  qDesired_SunPointing/1 -> Sun Pointing Algorithm (LQR)/4(Desired Quaternion [Sun Pointing])
  MeasuredMagneticField_Body/1 -> Sun Pointing Algorithm (LQR)/2(Measured Magnetic Field [Body] (T))
  Sun Pointing Algorithm (LQR)/3(Error Quaternion) -> ErrorQuaternion/1

== system ADCSSimulator/ADCS/ADCS Software/Attitude Control/Wheel Momentum Calculator ==
  Actuators Feedback : Inport
  Bus Selector : BusSelector  OutputSignals=RWs.RWs Angular Velocity [Body].RWs Angular Velocity (rad/s).RW#1 Motor Angular Velocity (rad/s),RWs.RWs Angular Velocity [Body].RWs Angular Velocity (rad/s).RW#2 Motor Angular Velocity (rad/s),RWs.RWs Angular Velocity [Body].RWs Angular Velocity (rad/s).RW#3 Motor Angular Velocity (rad/s)
  Gain : Gain  Gain=J
  Mux : Mux  Inputs=3
  Reshape : Reshape  OutputDimensionality=Column vector (2-D)
  Wheel Momentum Vector : Outport
  wires:
  Actuators Feedback/1 -> Bus Selector/1
  Bus Selector/1 -> Mux/1  "<RW#1 Motor Angular Velocity (rad/s)>"
  Bus Selector/2 -> Mux/2  "<RW#2 Motor Angular Velocity (rad/s)>"
  Bus Selector/3 -> Mux/3  "<RW#3 Motor Angular Velocity (rad/s)>"
  Reshape/1 -> Gain/1
  Gain/1 -> Wheel Momentum Vector/1
  Mux/1 -> Reshape/1

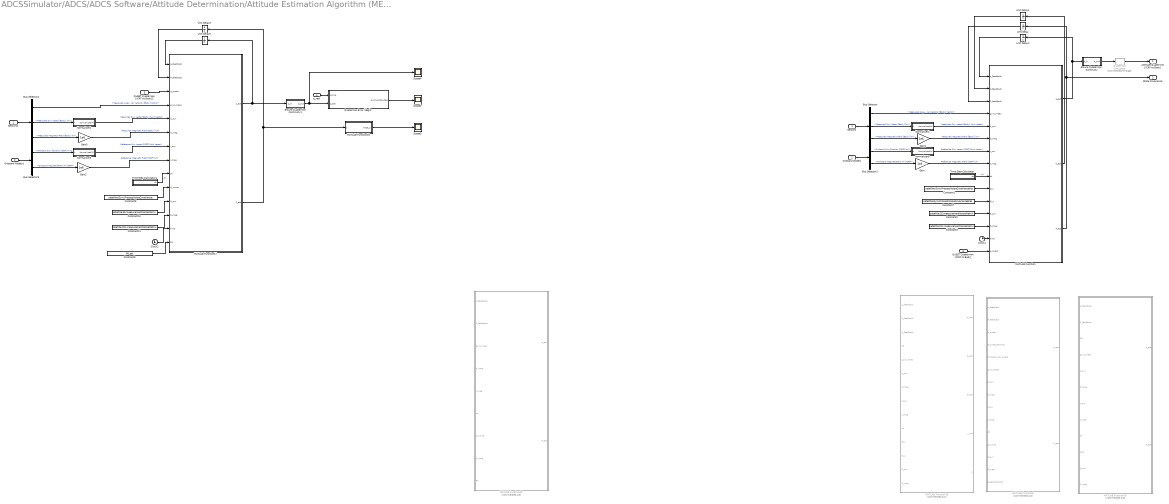
== system ADCSSimulator/ADCS/ADCS Software/Attitude Determination/Attitude Estimation Algorithm (MEKF) ==
  Sensors : Inport
  Onboard Models : Inport  Port=2
  QUEST Quaternion [ICRF to Body] : Inport  Port=3
  q_real : Inport  Port=4
  Bus Selector : BusSelector  OutputSignals=Measured Angular Velocity [Body] (rad/s),Measured Sun Vector [Body] (m),Measured Magnetic Field [Body] (T)
  Bus Selector1 : BusSelector  OutputSignals=|
      | Onboard Sun Ephemeris.Onboard Sun Position [ICRF] (m),Onboard Magnetic Field.Onboard MagneticField
      | (T) [ICRF]
  Bus Selector2 : BusSelector  OutputSignals=Measured Angular Velocity [Body] (rad/s),Measured Sun Vector [Body] (m),Measured Magnetic Field [Body] (T)
  Bus Selector3 : BusSelector  OutputSignals=|
      | Onboard Sun Ephemeris.Onboard Sun Position [ICRF] (m),Onboard Magnetic Field.Onboard MagneticField
      | (T) [ICRF]
  Clock1 : Clock
  Clock2 : Clock
  Constant1 : Constant  Value=satellite.Gyro.ProcessNoiseCovarianceAtt
  Constant10 : Constant  Value=satellite.SS.measurementNoiseMatrix
  Constant11 : Constant  Value=satellite.MM.measurementNoiseMatrix
  Constant2 : Constant  Value=satellite.SS.measurementNoiseMatrix
  Constant3 : Constant  Value=satellite.MM.measurementNoiseMatrix
  Constant5 : Constant  Value=satellite.Gyro.ProcessNoiseCovariance
  Constant7 : Constant  Value=satellite.Gyro.ProcessNoiseCovarianceBias
  Constant9 : Constant  Value=P0_att
  Ensure Quaternion Continuity : Subsystem
  Ensure Quaternion Continuity1 : Subsystem
  Gain{,1..3} (4 alike) : Gain  Gain=1e6
  MATLAB Function : MATLAB Function  TreatAsAtomicUnit=on
  MATLAB Function16 : MATLAB Function  Commented=on  TreatAsAtomicUnit=on
  MATLAB Function17 : MATLAB Function  TreatAsAtomicUnit=on
  MATLAB Function18 : MATLAB Function  Commented=on  TreatAsAtomicUnit=on
  MATLAB Function19 : MATLAB Function  TreatAsAtomicUnit=on
  MATLAB Function20 : MATLAB Function  Commented=on  TreatAsAtomicUnit=on
  MATLAB Function9 : MATLAB Function  Commented=on  TreatAsAtomicUnit=on
  Normalizer1 : Subsystem
  Normalizer2 : Subsystem
  Normalizer3 : Subsystem
  Normalizer8 : Subsystem
  Onboard Models1 : InportShadow  Port=2
  QUEST Quaternion [ICRF to Body]2 : InportShadow  Port=3
  Quaternion Conjugate : aerolibutil/Quaternion Conjugate  Commented=through
  Quaternion Error (deg)2 : MATLAB Function  TreatAsAtomicUnit=on
  Scope2 : Scope
  Scope3 : Scope
  Scope4 : Scope
  Sensors1 : InportShadow
  Time Step Calculator : Subsystem
  Time Step Calculator1 : Subsystem
  Unit Delay : UnitDelay  InitialCondition=P0  SampleTime=-1  HasFrameUpgradeWarning=on
  Unit Delay1 : UnitDelay  InitialCondition=zeros(3,1)  SampleTime=-1  HasFrameUpgradeWarning=on
  Unit Delay2 : UnitDelay  InitialCondition=[1;0;0;0]  SampleTime=-1  HasFrameUpgradeWarning=on
  Unit Delay3 : UnitDelay  InitialCondition=P0_att  SampleTime=-1  HasFrameUpgradeWarning=on
  Unit Delay5 : UnitDelay  InitialCondition=[1;0;0;0]  SampleTime=-1  HasFrameUpgradeWarning=on
  Attitude Quaternion [ICRF to Body] : Outport
  State Covariance : Outport  Port=2
  wires:
  Ensure Quaternion Continuity/1(q_out) -> Quaternion Conjugate/1
  Bus Selector1/1 -> Normalizer8/1(A)  "<Onboard Sun Position [ICRF] (m)>"
  MATLAB Function/1(q_est) -> Unit Delay2/1, Ensure Quaternion Continuity/1(q_in)
  Bus Selector/2 -> Normalizer1/1(A)  "<Measured Sun Vector [Body] (m)>"
  Bus Selector1/2 -> Gain/1  "<Onboard MagneticField (T) [ICRF]>"
  Onboard Models/1 -> Bus Selector1/1
  Time Step Calculator/1(dt) -> MATLAB Function/9(dt)  "dt"
  Unit Delay/1 -> MATLAB Function/3(P_feedback)
  Bus Selector/1 -> MATLAB Function/4(gyro_meas)  "<Measured Angular Velocity [Body] (rad/s)>"
  Sensors/1 -> Bus Selector/1
  Constant3/1 -> MATLAB Function/13(R_mag)
  Constant2/1 -> MATLAB Function/12(R_sun)
  Bus Selector/3 -> Gain1/1  "<Measured Magnetic Field [Body] (T)>"
  Unit Delay2/1 -> MATLAB Function/1(q_feedback)
  Gain/1 -> MATLAB Function/8(r_mag)  "Reference Magnetic Field [ICRF] (uT)"
  Gain1/1 -> MATLAB Function/6(b_mag)  "Measured Magnetic Field [Body] (uT)"
  Normalizer8/1(Normalized(A)) -> MATLAB Function/7(r_sun)  "Reference Sun Vector [ICRF] (Unit Vector)"
  Normalizer1/1(Normalized(A)) -> MATLAB Function/5(b_sun)  "Measured Sun Vector [Body] (Unit Vector)"
  QUEST Quaternion [ICRF to Body]/1 -> MATLAB Function/15(q_quest)
  MATLAB Function/2(b_est) -> Unit Delay1/1
  Unit Delay1/1 -> MATLAB Function/2(b_feedback)
  Constant7/1 -> MATLAB Function/11(Q_u)
  Constant1/1 -> MATLAB Function/10(Q_v)
  Clock1/1 -> MATLAB Function/14(time)
  Constant5/1 -> MATLAB Function17/10(Q_noise)
  Time Step Calculator1/1(dt) -> MATLAB Function17/9(dt)  "dt"
  Constant10/1 -> MATLAB Function17/11(R_sun)
  Clock2/1 -> MATLAB Function17/13(time)
  Constant11/1 -> MATLAB Function17/12(R_mag)
  Unit Delay3/1 -> MATLAB Function17/2(P_feedback)
  Normalizer3/1(Normalized(A)) -> MATLAB Function17/7(r_sun)  "Reference Sun Vector [ICRF] (Unit Vector)"
  Bus Selector3/2 -> Gain2/1  "<Onboard MagneticField (T) [ICRF]>"
  Normalizer2/1(Normalized(A)) -> MATLAB Function17/5(b_sun)  "Measured Sun Vector [Body] (Unit Vector)"
  QUEST Quaternion [ICRF to Body]2/1 -> MATLAB Function17/3(q_quest)
  Gain3/1 -> MATLAB Function17/6(b_mag)  "Measured Magnetic Field [Body] (uT)"
  Unit Delay5/1 -> MATLAB Function17/1(q_feedback)
  Bus Selector2/3 -> Gain3/1  "<Measured Magnetic Field [Body] (T)>"
  MATLAB Function17/1(q_est) -> Ensure Quaternion Continuity1/1(q_in), Unit Delay5/1
  Bus Selector2/1 -> MATLAB Function17/4(gyro_meas)  "<Measured Angular Velocity [Body] (rad/s)>"
  MATLAB Function17/2(P_est) -> Unit Delay3/1, MATLAB Function19/1(p)
  Bus Selector2/2 -> Normalizer2/1(A)  "<Measured Sun Vector [Body] (m)>"
  Bus Selector3/1 -> Normalizer3/1(A)  "<Onboard Sun Position [ICRF] (m)>"
  Gain2/1 -> MATLAB Function17/8(r_mag)  "Reference Magnetic Field [ICRF] (uT)"
  Onboard Models1/1 -> Bus Selector3/1
  Sensors1/1 -> Bus Selector2/1
  MATLAB Function19/1(trace_p) -> Scope3/1
  Ensure Quaternion Continuity1/1(q_out) -> Scope4/1, Quaternion Error (deg)2/2(q_est)
  q_real/1 -> Quaternion Error (deg)2/1(q_true)
  Quaternion Error (deg)2/1(error_angle_deg) -> Scope2/1
  Constant9/1 -> MATLAB Function17/14(P0)
  Quaternion Conjugate/1 -> Attitude Quaternion [ICRF to Body]/1
  MATLAB Function/3(P_est) -> State Covariance/1, Unit Delay/1

== system ADCSSimulator/ADCS/ADCS Software/Attitude Determination/Static Attitude Determination Algorithm (QUEST) ==
  Sensors Data : Inport
  Onboard Models : Inport  Port=2
  Bus Selector : BusSelector  OutputSignals=|
      | Onboard Sun Ephemeris.Onboard Sun Position [ICRF] (m),Onboard Magnetic Field.Onboard MagneticField
      | (T) [ICRF]
  Bus Selector1 : BusSelector  OutputSignals=Measured Sun Vector [Body] (m),Measured Magnetic Field [Body] (T)
  Constant10 : Constant  Value=0.65
  Constant11 : Constant  Value=0.35
  Ensure Quaternion Continuity1 : Subsystem
  Static Attitude Determination Algorithm (QUEST) : MATLAB Function  TreatAsAtomicUnit=on
  Unit Delay5 : UnitDelay  InitialCondition=[1;0;0;0]  SampleTime=-1  HasFrameUpgradeWarning=on
  QUEST: Covariance Matrix : Outport
  QUEST: lambda_max : Outport  Port=2
  QUEST: ICRF to Body Quaternion : Outport  Port=3
  wires:
  Static Attitude Determination Algorithm (QUEST)/1(q) -> Unit Delay5/1, Ensure Quaternion Continuity1/1(q_in)
  Unit Delay5/1 -> Static Attitude Determination Algorithm (QUEST)/7(q_prev)
  Constant11/1 -> Static Attitude Determination Algorithm (QUEST)/6(w_mag)
  Constant10/1 -> Static Attitude Determination Algorithm (QUEST)/5(w_sun)
  Bus Selector1/2 -> Static Attitude Determination Algorithm (QUEST)/4(b_mag)  "<Measured Magnetic Field [Body] (T)>"
  Onboard Models/1 -> Bus Selector/1
  Bus Selector1/1 -> Static Attitude Determination Algorithm (QUEST)/3(b_sun)  "<Measured Sun Vector [Body] (m)>"
  Bus Selector/1 -> Static Attitude Determination Algorithm (QUEST)/1(r_sun)  "<Onboard Sun Position [ICRF] (m)>"
  Sensors Data/1 -> Bus Selector1/1
  Bus Selector/2 -> Static Attitude Determination Algorithm (QUEST)/2(r_mag)  "<Onboard MagneticField (T) [ICRF]>"
  Static Attitude Determination Algorithm (QUEST)/2(P) -> QUEST: Covariance Matrix/1
  Static Attitude Determination Algorithm (QUEST)/3(lambda_max) -> QUEST: lambda_max/1
  Ensure Quaternion Continuity1/1(q_out) -> QUEST: ICRF to Body Quaternion/1

== system ADCSSimulator/ADCS/ADCS Software/Attitude Guidance/Normalizer5 ==
  A : Inport
  Divide : Product  Inputs=*/
  Dot Product : DotProduct  OutDataTypeStr=Inherit: Inherit via internal rule
  Sqrt1 : Sqrt
  Normalized(A) : Outport
  wires:
  Divide/1 -> Normalized(A)/1
  Sqrt1/1 -> Divide/2
  A/1 -> Dot Product/1, Dot Product/2, Divide/1
  Dot Product/1 -> Sqrt1/1

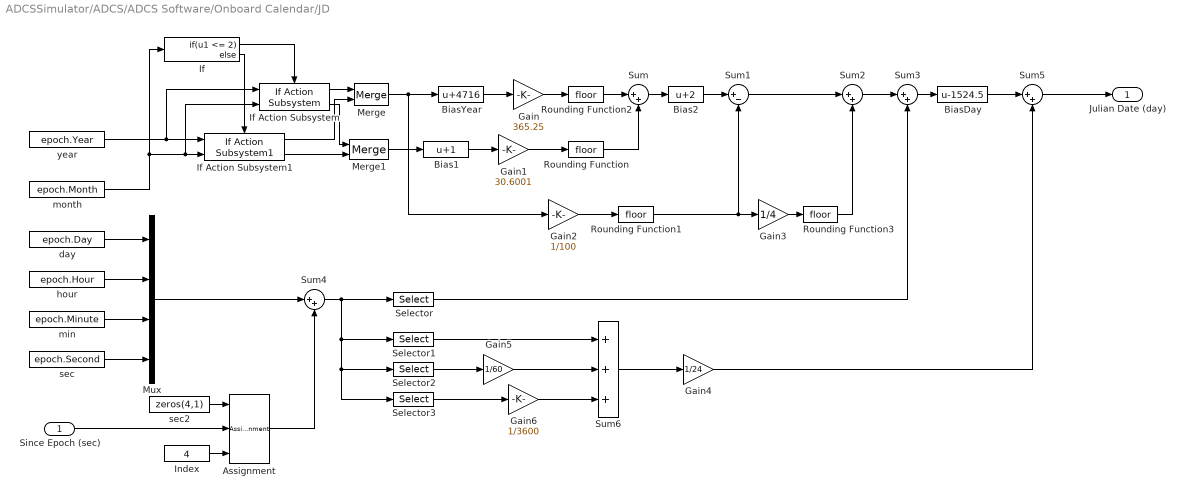
== system ADCSSimulator/ADCS/ADCS Software/Onboard Calendar/JD ==
  Since Epoch (sec) : Inport  OutMin=0  PortDimensions=1
  Assignment : Assignment  IndexOptions=Index vector (port)  Indices=1  OutputSizes=1
  Bias1 : Bias  Bias=1  SaturateOnIntegerOverflow=off
  Bias2 : Bias  Bias=2  SaturateOnIntegerOverflow=off
  BiasDay : Bias  Bias=-1524.5  SaturateOnIntegerOverflow=off
  BiasYear : Bias  Bias=4716  SaturateOnIntegerOverflow=off
  Gain : Gain  Gain=365.25
  Gain1 : Gain  Gain=30.6001
  Gain2 : Gain  Gain=1/100
  Gain3 : Gain  Gain=1/4
  Gain4 : Gain  Gain=1/24
  Gain5 : Gain  Gain=1/60
  Gain6 : Gain  Gain=1/3600
  If : If  IfExpression=u1 <= 2
  If Action Subsystem : aerolibconvert2/Julian Date Conversion/If Action Subsystem  SystemSampleTime=-1  VariantActivationTime=update diagram  AllowFlexibleInterface=on  Latency=0  AutoFrameSizeCalculation=off
  If Action Subsystem1 : aerolibconvert2/Julian Date Conversion/If Action Subsystem1  SystemSampleTime=-1  VariantActivationTime=update diagram  AllowFlexibleInterface=on  Latency=0  AutoFrameSizeCalculation=off
  Index : Constant  Value=4
  Merge : Merge
  Merge1 : Merge
  Mux : Mux
  Rounding Function{,1..3} (4 alike) : Rounding
  Selector : Selector  InputPortWidth=4  IndexOptions=Index vector (dialog)  Indices=[1]  OutputSizes=1
  Selector1 : Selector  InputPortWidth=4  IndexOptions=Index vector (dialog)  Indices=[2]  OutputSizes=1
  Selector2 : Selector  InputPortWidth=4  IndexOptions=Index vector (dialog)  Indices=[3]  OutputSizes=1
  Selector3 : Selector  InputPortWidth=4  IndexOptions=Index vector (dialog)  Indices=[4]  OutputSizes=1
  Sum{,2..5} (5 alike) : Sum  Inputs=|++
  Sum1 : Sum  Inputs=|+-
  Sum6 : Sum  Inputs=+++
  day : Constant  Value=epoch.Day
  hour : Constant  Value=epoch.Hour
  min : Constant  Value=epoch.Minute
  month : Constant  Value=epoch.Month
  sec : Constant  Value=epoch.Second
  sec2 : Constant  Value=zeros(4,1)
  year : Constant  Value=epoch.Year
  Julian Date (day) : Outport  VectorParamsAs1DForOutWhenUnconnected=off
  wires:
  Merge1/1 -> Bias1/1
  Mux/1 -> Sum4/1
  month/1 -> If/1, If Action Subsystem1/2, If Action Subsystem/2
  Rounding Function/1 -> Sum/2
  day/1 -> Mux/1
  If Action Subsystem1/2 -> Merge1/2
  Sum/1 -> Bias2/1
  Sum6/1 -> Gain4/1
  BiasDay/1 -> Sum5/1
  hour/1 -> Mux/2
  Selector/1 -> Sum3/2
  sec/1 -> Mux/4
  Since Epoch (sec)/1 -> Assignment/2
  If/2 -> If Action Subsystem1/Action
  Rounding Function1/1 -> Sum1/2, Gain3/1
  Gain5/1 -> Sum6/2
  Assignment/1 -> Sum4/2
  Bias2/1 -> Sum1/1
  Gain/1 -> Rounding Function2/1
  Gain2/1 -> Rounding Function1/1
  Sum4/1 -> Selector/1, Selector3/1, Selector2/1, Selector1/1
  If Action Subsystem/1 -> Merge/1
  year/1 -> If Action Subsystem1/1, If Action Subsystem/1
  Gain6/1 -> Sum6/3
  Sum3/1 -> BiasDay/1
  If Action Subsystem/2 -> Merge1/1
  Bias1/1 -> Gain1/1
  Rounding Function3/1 -> Sum2/2
  Gain1/1 -> Rounding Function/1
  sec2/1 -> Assignment/1
  Sum1/1 -> Sum2/1
  Sum5/1 -> Julian Date (day)/1
  Selector1/1 -> Sum6/1
  Sum2/1 -> Sum3/1
  Gain4/1 -> Sum5/2
  BiasYear/1 -> Gain/1
  Merge/1 -> BiasYear/1, Gain2/1
  Gain3/1 -> Rounding Function3/1
  Selector2/1 -> Gain5/1
  Rounding Function2/1 -> Sum/1
  Selector3/1 -> Gain6/1
  If/1 -> If Action Subsystem/Action
  min/1 -> Mux/3
  If Action Subsystem1/1 -> Merge/2
  Index/1 -> Assignment/3

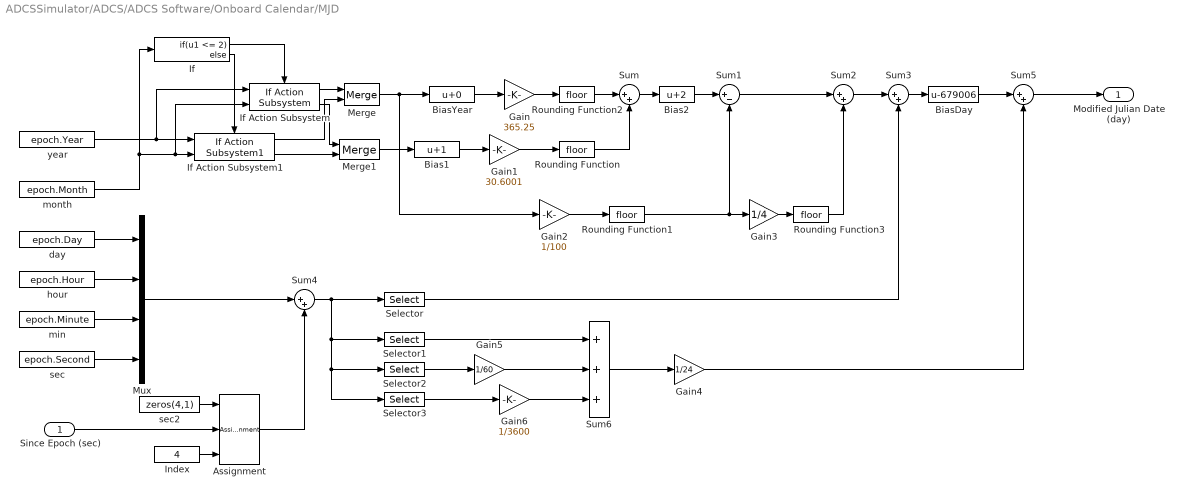
== system ADCSSimulator/ADCS/ADCS Software/Onboard Calendar/MJD ==
  Since Epoch (sec) : Inport  OutMin=0  PortDimensions=1
  Assignment : Assignment  IndexOptions=Index vector (port)  Indices=1  OutputSizes=1
  Bias1 : Bias  Bias=1  SaturateOnIntegerOverflow=off
  Bias2 : Bias  Bias=2  SaturateOnIntegerOverflow=off
  BiasDay : Bias  Bias=-679006  SaturateOnIntegerOverflow=off
  BiasYear : Bias  SaturateOnIntegerOverflow=off
  Gain : Gain  Gain=365.25
  Gain1 : Gain  Gain=30.6001
  Gain2 : Gain  Gain=1/100
  Gain3 : Gain  Gain=1/4
  Gain4 : Gain  Gain=1/24
  Gain5 : Gain  Gain=1/60
  Gain6 : Gain  Gain=1/3600
  If : If  IfExpression=u1 <= 2
  If Action Subsystem : aerolibconvert2/Julian Date Conversion/If Action Subsystem  SystemSampleTime=-1  VariantActivationTime=update diagram  AllowFlexibleInterface=on  Latency=0  AutoFrameSizeCalculation=off
  If Action Subsystem1 : aerolibconvert2/Julian Date Conversion/If Action Subsystem1  SystemSampleTime=-1  VariantActivationTime=update diagram  AllowFlexibleInterface=on  Latency=0  AutoFrameSizeCalculation=off
  Index : Constant  Value=4
  Merge : Merge
  Merge1 : Merge
  Mux : Mux
  Rounding Function{,1..3} (4 alike) : Rounding
  Selector : Selector  InputPortWidth=4  IndexOptions=Index vector (dialog)  Indices=[1]  OutputSizes=1
  Selector1 : Selector  InputPortWidth=4  IndexOptions=Index vector (dialog)  Indices=[2]  OutputSizes=1
  Selector2 : Selector  InputPortWidth=4  IndexOptions=Index vector (dialog)  Indices=[3]  OutputSizes=1
  Selector3 : Selector  InputPortWidth=4  IndexOptions=Index vector (dialog)  Indices=[4]  OutputSizes=1
  Sum{,2..5} (5 alike) : Sum  Inputs=|++
  Sum1 : Sum  Inputs=|+-
  Sum6 : Sum  Inputs=+++
  day : Constant  Value=epoch.Day
  hour : Constant  Value=epoch.Hour
  min : Constant  Value=epoch.Minute
  month : Constant  Value=epoch.Month
  sec : Constant  Value=epoch.Second
  sec2 : Constant  Value=zeros(4,1)
  year : Constant  Value=epoch.Year
  Modified Julian Date (day) : Outport  VectorParamsAs1DForOutWhenUnconnected=off
  wires:
  Rounding Function/1 -> Sum/2
  If/2 -> If Action Subsystem1/Action
  Gain4/1 -> Sum5/2
  BiasYear/1 -> Gain/1
  Bias2/1 -> Sum1/1
  Selector1/1 -> Sum6/1
  Sum/1 -> Bias2/1
  Sum2/1 -> Sum3/1
  BiasDay/1 -> Sum5/1
  Selector/1 -> Sum3/2
  Sum1/1 -> Sum2/1
  year/1 -> If Action Subsystem1/1, If Action Subsystem/1
  Sum5/1 -> Modified Julian Date (day)/1
  Sum6/1 -> Gain4/1
  hour/1 -> Mux/2
  Gain/1 -> Rounding Function2/1
  Merge1/1 -> Bias1/1
  Since Epoch (sec)/1 -> Assignment/2
  Gain6/1 -> Sum6/3
  Gain2/1 -> Rounding Function1/1
  Mux/1 -> Sum4/1
  Rounding Function1/1 -> Sum1/2, Gain3/1
  Rounding Function3/1 -> Sum2/2
  Sum3/1 -> BiasDay/1
  Selector3/1 -> Gain6/1
  Rounding Function2/1 -> Sum/1
  Gain1/1 -> Rounding Function/1
  sec2/1 -> Assignment/1
  day/1 -> Mux/1
  Bias1/1 -> Gain1/1
  min/1 -> Mux/3
  Gain3/1 -> Rounding Function3/1
  If/1 -> If Action Subsystem/Action
  Gain5/1 -> Sum6/2
  If Action Subsystem1/1 -> Merge/2
  Sum4/1 -> Selector/1, Selector3/1, Selector2/1, Selector1/1
  Merge/1 -> BiasYear/1, Gain2/1
  If Action Subsystem/1 -> Merge/1
  Selector2/1 -> Gain5/1
  If Action Subsystem/2 -> Merge1/1
  month/1 -> If/1, If Action Subsystem1/2, If Action Subsystem/2
  sec/1 -> Mux/4
  If Action Subsystem1/2 -> Merge1/2
  Assignment/1 -> Sum4/2
  Index/1 -> Assignment/3

== system ADCSSimulator/ADCS/ADCS Software/Onboard Calendar/Time Step Calculator ==
  Clock : Clock
  Sum : Sum  Inputs=|+-
  Unit Delay3 : UnitDelay  SampleTime=-1  HasFrameUpgradeWarning=on
  dt : Outport
  wires:
  Clock/1 -> Sum/1, Unit Delay3/1
  Unit Delay3/1 -> Sum/2
  Sum/1 -> dt/1

== system ADCSSimulator/ADCS/ADCS Software/Onboard Models/Onboard Sun Ephemeris Calculator ==
  Onboard Calendar : Inport
  Bus Selector : BusSelector  OutputSignals=Julian Date (day)
  Length Conversion1 : aerolibconvert2/Length Conversion  IU=km  OU=m
  Sun Ephemeris Bus Creator : BusCreator  Inputs=2
  Sun Ephemeris Calculator : PlanetaryEphem  target=Sun
  Velocity Conversion1 : aerolibconvert2/Velocity Conversion  IU=km/s  OU=m/s
  Onboard Sun Ephemeris [ICRF] : Outport
  wires:
  Sun Ephemeris Bus Creator/1 -> Onboard Sun Ephemeris [ICRF]/1  "Onboard Sun Ephemeris [ICRF]"
  Length Conversion1/1 -> Sun Ephemeris Bus Creator/1  "Onboard Sun Position [ICRF] (m)"
  Sun Ephemeris Calculator/2 -> Velocity Conversion1/1
  Sun Ephemeris Calculator/1 -> Length Conversion1/1
  Velocity Conversion1/1 -> Sun Ephemeris Bus Creator/2  "Onboard Sun Velocity [ICRF] (m/s)"
  Onboard Calendar/1 -> Bus Selector/1
  Bus Selector/1 -> Sun Ephemeris Calculator/1  "<Julian Date (day)>"

== system ADCSSimulator/ADCS/ADCS Software/Onboard Models/WMM ==
  Satellite Position [ICRF] (m) : Inport
  Calendar : Inport  Port=2
  Transformers : Inport  Port=3
  Bus Selector : BusSelector  OutputSignals=Decimal Year (year)
  Bus Selector2 : BusSelector  OutputSignals=Transfer Matrices.ICRF to ITRF TM
  Bus Selector4 : BusSelector  OutputSignals=Transfer Matrices.ICRF to ITRF TM
  Convert to Teslla : Gain  Gain=10^-9  Multiplication=Matrix(K*u)
  Demux : Demux  Outputs=2
  Direction Cosine Matrix ECEF to NED : aerolibtransform2/Direction Cosine Matrix ECEF to NED
  Divide : Product  Inputs=**  Multiplication=Matrix(*)
  Divide2 : Product  Inputs=**  Multiplication=Matrix(*)
  Divide3 : Product  Inputs=**  Multiplication=Matrix(*)
  ECEF Position to LLA : ECEF2LLA
  Mux : Mux  Inputs=2
  Onboard Magnetic Field Bus Creator : BusCreator  Inputs=2
  Reshape : Reshape  OutputDimensionality=Customize  OutputDimensions=[3,1]
  Transpose : Math  Operator=transpose
  Transpose1 : Math  Operator=transpose
  World Magnetic Model : aerolibgravity2/World Magnetic Model  model=WMM2020 (2020-2025)  customFile='WMM2020.COF'  units=Metric (MKS)  time_in=on  month=January  day=1  year=2020  action=Error  h_out=off  dec_out=off  inc_out=off  ti_out=off
  Onboard Magnetic Field (T) : Outport
  wires:
  [Latitude_deg] -> World Magnetic Model/2  "Latitude (deg)"
  Transpose/1 -> Divide/1
  Demux/1 -> [Latitude_deg]
  [Altitude_m] -> World Magnetic Model/1  "Altitude (m)"
  Reshape/1 -> Divide3/2, Onboard Magnetic Field Bus Creator/2  "Onboard Magnetic Field (T) [ITRF]"
  Direction Cosine Matrix ECEF to NED/1 -> Transpose/1
  Onboard Magnetic Field Bus Creator/1 -> Onboard Magnetic Field (T)/1  "Onboard Magnetic Field (T)"
  Mux/1 -> Direction Cosine Matrix ECEF to NED/1
  Transformers/1 -> Bus Selector4/1, Bus Selector2/1
  [Latitude_deg] -> Mux/1  "Latitude (deg)"
  [Longitude_deg] -> Mux/2  "Longitude (deg)"
  ECEF Position to LLA/2 -> [Altitude_m]
  Demux/2 -> [Longitude_deg]
  Divide/1 -> Convert to Teslla/1
  Convert to Teslla/1 -> Reshape/1
  Calendar/1 -> Bus Selector/1
  ECEF Position to LLA/1 -> Demux/1
  Divide2/1 -> ECEF Position to LLA/1  "Satellite Position [ITRF] (m)"
  [Longitude_deg] -> World Magnetic Model/3  "Longitude (deg)"
  Bus Selector/1 -> World Magnetic Model/4  "<Decimal Year (year)>"
  World Magnetic Model/1 -> Divide/2
  Bus Selector2/1 -> Divide2/1  "<ICRF to ITRF TM>"
  Satellite Position [ICRF] (m)/1 -> Divide2/2
  Bus Selector4/1 -> Transpose1/1  "<ICRF to ITRF TM>"
  Transpose1/1 -> Divide3/1  "ITRF to ICRF TM"
  Divide3/1 -> Onboard Magnetic Field Bus Creator/1  "Onboard MagneticField (T) [ICRF]"

== system ADCSSimulator/ADCS/ADCS Software/Onboard Reference Frames Transformations Manager1/Ensure Quaternion Continuity ==
  q_in : Inport
  Ensure Quaternion Continuity : MATLAB Function  TreatAsAtomicUnit=on
  Unit Delay : UnitDelay  InitialCondition=[1;0;0;0]  SampleTime=-1  HasFrameUpgradeWarning=on
  q_out : Outport
  wires:
  Ensure Quaternion Continuity/1(q_out) -> q_out/1, Unit Delay/1
  Unit Delay/1 -> Ensure Quaternion Continuity/2(q_prev)
  q_in/1 -> Ensure Quaternion Continuity/1(q_new)

== system ADCSSimulator/ADCS/ADCS Software/Onboard Reference Frames Transformations Manager1/Ensure Quaternion Continuity1 ==
  q_in : Inport
  Ensure Quaternion Continuity : MATLAB Function  TreatAsAtomicUnit=on
  Unit Delay : UnitDelay  InitialCondition=[1;0;0;0]  SampleTime=-1  HasFrameUpgradeWarning=on
  q_out : Outport
  wires:
  Ensure Quaternion Continuity/1(q_out) -> q_out/1, Unit Delay/1
  Unit Delay/1 -> Ensure Quaternion Continuity/2(q_prev)
  q_in/1 -> Ensure Quaternion Continuity/1(q_new)

== system ADCSSimulator/ADCS/ADCS Software/Onboard Reference Frames Transformations Manager1/Ensure Quaternion Continuity2 ==
  q_in : Inport
  Ensure Quaternion Continuity : MATLAB Function  TreatAsAtomicUnit=on
  Unit Delay : UnitDelay  InitialCondition=[1;0;0;0]  SampleTime=-1  HasFrameUpgradeWarning=on
  q_out : Outport
  wires:
  Ensure Quaternion Continuity/1(q_out) -> q_out/1, Unit Delay/1
  Unit Delay/1 -> Ensure Quaternion Continuity/2(q_prev)
  q_in/1 -> Ensure Quaternion Continuity/1(q_new)
